simulink model "hovercraft_kinematic_control"  (R2024a)
settings: Solver=VariableStepAuto  StartTime=0.0  StopTime=20  RelTol=1e-3
settings Model: Creator=ettor  LastModifiedBy=ettor

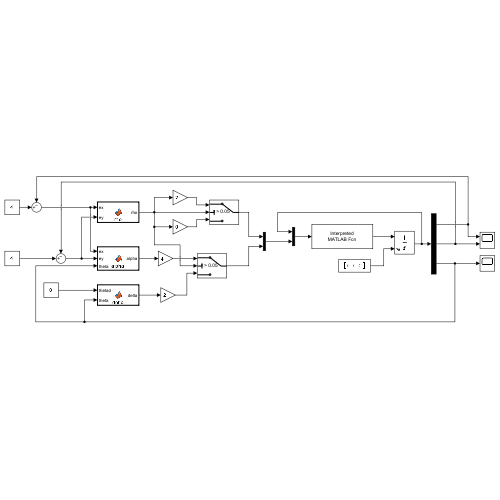
[thumbnail: Simulink's stored preview of the top-level diagram]
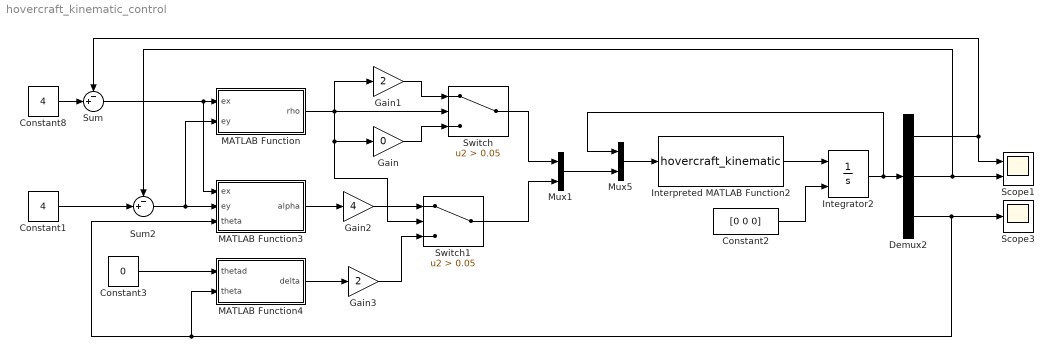
== system hovercraft_kinematic_control ==
  Constant1 : Constant  Value=4
  Constant2 : Constant  Value=[0 0 0]
  Constant3 : Constant  Value=0
  Constant8 : Constant  Value=4
  Demux2 : Demux  Outputs=3
  Gain : Gain  Gain=0
  Gain1 : Gain  Gain=2
  Gain2 : Gain  Gain=4
  Gain3 : Gain  Gain=2
  Integrator2 : Integrator  InitialConditionSource=external
  Interpreted MATLAB Function2 : MATLABFcn  MATLABFcn=hovercraft_kinematic
  MATLAB Function : MATLAB Function  TreatAsAtomicUnit=on
  MATLAB Function3 : MATLAB Function  TreatAsAtomicUnit=on
  MATLAB Function4 : MATLAB Function  TreatAsAtomicUnit=on
  Mux1 : Mux  Inputs=2
  Mux5 : Mux  Inputs=2
  Scope1 : Scope  NumInputPorts=2
  Scope3 : Scope
  Sum : Sum  Inputs=-+|
  Sum2 : Sum  Inputs=-+|
  Switch : Switch  Criteria=u2 > Threshold  Threshold=0.05  SaturateOnIntegerOverflow=off  InputSameDT=off
  Switch1 : Switch  Criteria=u2 > Threshold  Threshold=0.05  SaturateOnIntegerOverflow=off  InputSameDT=off
  wires:
  Sum/1 -> MATLAB Function/1(ex), MATLAB Function3/1(ex)
  Constant8/1 -> Sum/2
  MATLAB Function/1(rho) -> Gain1/1, Switch/2, Switch1/2, Gain/1
  MATLAB Function4/1(delta) -> Gain3/1
  Switch/1 -> Mux1/1
  MATLAB Function3/1(alpha) -> Gain2/1
  Constant3/1 -> MATLAB Function4/1(thetad)
  Gain3/1 -> Switch1/3
  Gain/1 -> Switch/3
  Demux2/3 -> Scope3/1, MATLAB Function4/2(theta), MATLAB Function3/3(theta)
  Switch1/1 -> Mux1/2
  Gain2/1 -> Switch1/1
  Integrator2/1 -> Mux5/1, Demux2/1
  Demux2/2 -> Scope1/2, Sum2/1
  Gain1/1 -> Switch/1
  Constant2/1 -> Integrator2/2
  Mux1/1 -> Mux5/2
  Constant1/1 -> Sum2/2
  Demux2/1 -> Sum/1, Scope1/1
  Mux5/1 -> Interpreted MATLAB Function2/1
  Sum2/1 -> MATLAB Function/2(ey), MATLAB Function3/2(ey)
  Interpreted MATLAB Function2/1 -> Integrator2/1

== matlab function hovercraft_kinematic_control/MATLAB Function3 ==
  data: ex input; alpha output; ey input; theta input
function alpha = alpha(ex,ey,theta)
    alpha = atan2(ey, ex) - theta;
    alpha = atan2(sin(alpha), cos(alpha));
end

== matlab function hovercraft_kinematic_control/MATLAB Function4 ==
  data: thetad input; delta output; theta input
function delta = delta(thetad,theta)
    delta = thetad - theta;
    delta = atan2(sin(delta), cos(delta));
end

== matlab function hovercraft_kinematic_control/MATLAB Function ==
  data: ex input; rho output; ey input
function rho = rho(ex,ey)
    rho = sqrt(ex^2 + ey^2);
end
